simulink model "das_model"  (R2026a)
settings: Solver=FixedStepDiscrete  StopTime=T_sim  FixedStep=Ts_slow
InitFcn:
  | addpath(fullfile(fileparts(get_param(bdroot,'FileName')),'..','scripts')); p = otdr_params(); das_init
undefined symbols (not defined in the file): att, B_cell, f_v, g_cir, g_edfa, g_vib, k_lo, k_sig, Ns, p, p_frame, P_laser, Phi0, r, R_pd, sigma_n_coh, sigma_n_dd, Ts_slow, var_phL
settings Model: Creator=aljou  LastModifiedBy=aljou

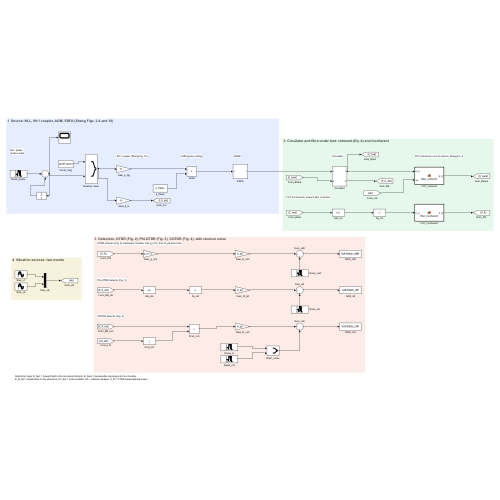
[thumbnail: Simulink's stored preview of the top-level diagram]
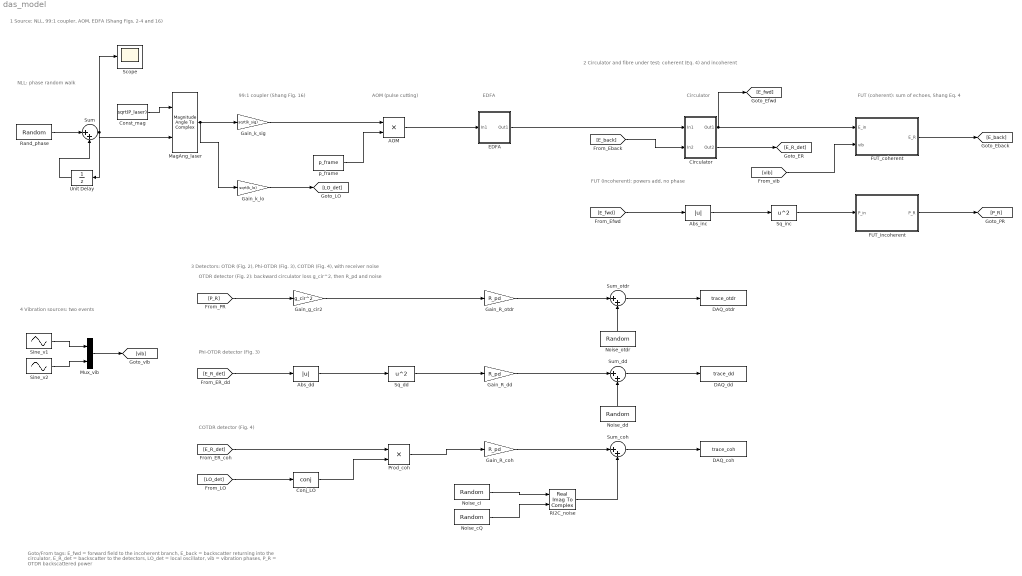
== system das_model ==
  note: NLL: phase
      | random walk
  note: 99:1 coupler (Shang Fig. 16)
  note: AOM (pulse cutting)
  note: EDFA
  note: Circulator
  note: FUT (coherent): sum of echoes, Shang Eq. 4
  note: FUT (incoherent): powers add, no phase
  note: OTDR detector (Fig. 2): backward circulator loss g_cir^2, then R_pd and noise
  note: Phi-OTDR detector (Fig. 3)
  note: COTDR detector (Fig. 4)
  note: Goto/From tags: E_fwd = forward field to the incoherent branch, E_back = backscatter returning into the circulator,
      | E_R_det = backscatter to the detectors, LO_det = local oscillator, vib = vibration phases, P_R = OTDR backscattered power
  note: 1 Source: NLL, 99:1 coupler, AOM, EDFA (Shang Figs. 2-4 and 16)
  note: 2 Circulator and fibre under test: coherent (Eq. 4) and incoherent
  note: 3 Detectors: OTDR (Fig. 2), Phi-OTDR (Fig. 3), COTDR (Fig. 4), with receiver noise
  note: 4 Vibration sources: two events
  AOM : Product  Inputs=**
  Abs_dd : Abs  SaturateOnIntegerOverflow=off
  Abs_inc : Abs  SaturateOnIntegerOverflow=off
  Circulator : Subsystem
  Conj_LO : Math  Operator=conj
  Const_mag : Constant  Value=sqrt(P_laser)  SampleTime=Ts_slow
  DAQ_coh : ToWorkspace  VariableName=trace_coh  SampleTime=Ts_slow
  DAQ_dd : ToWorkspace  VariableName=trace_dd  SampleTime=Ts_slow
  DAQ_otdr : ToWorkspace  VariableName=trace_otdr  SampleTime=Ts_slow
  EDFA : Subsystem
  FUT_coherent : MATLAB Function  TreatAsAtomicUnit=on
  FUT_incoherent : MATLAB Function  TreatAsAtomicUnit=on
  Gain_R_coh : Gain  Gain=R_pd
  Gain_R_dd : Gain  Gain=R_pd
  Gain_R_otdr : Gain  Gain=R_pd
  Gain_g_cir2 : Gain  Gain=g_cir^2
  Gain_k_lo : Gain  Gain=sqrt(k_lo)
  Gain_k_sig : Gain  Gain=sqrt(k_sig)
  MagAng_laser : MagnitudeAngleToComplex
  Mux_vib : Mux  Inputs=2
  Noise_cI : RandomNumber  Mean=zeros(Ns,1)  Variance=sigma_n_coh^2  Seed=p.seed_noise(3)+(1:Ns).'  SampleTime=Ts_slow  VectorParams1D=off
  Noise_cQ : RandomNumber  Mean=zeros(Ns,1)  Variance=sigma_n_coh^2  Seed=p.seed_noise(4)+(1:Ns).'  SampleTime=Ts_slow  VectorParams1D=off
  Noise_dd : RandomNumber  Mean=zeros(Ns,1)  Variance=sigma_n_dd^2  Seed=p.seed_noise(2)+(1:Ns).'  SampleTime=Ts_slow  VectorParams1D=off
  Noise_otdr : RandomNumber  Mean=zeros(Ns,1)  Variance=sigma_n_dd^2  Seed=p.seed_noise(1)+(1:Ns).'  SampleTime=Ts_slow  VectorParams1D=off
  Prod_coh : Product  Inputs=**
  RI2C_noise : RealImagToComplex
  Rand_phase : RandomNumber  Variance=var_phL  Seed=p.seed_laser  SampleTime=Ts_slow
  Scope : Scope
      settings: ActiveDisplayYMinimum=-56.44665138784287  ActiveDisplayYMaximum=140.2998758824863
  Sine_v1 : Sin  Amplitude=Phi0(1)  Frequency=2*pi*f_v(1)  Phase=p.sine_phase  SampleTime=Ts_slow
  Sine_v2 : Sin  Amplitude=Phi0(2)  Frequency=2*pi*f_v(2)  Phase=p.sine_phase  SampleTime=Ts_slow
  Sq_dd : Math  Operator=square
  Sq_inc : Math  Operator=square
  Sum : Sum  Inputs=|++
  Sum_coh : Sum  Inputs=|++
  Sum_dd : Sum  Inputs=|++
  Sum_otdr : Sum  Inputs=|++
  Unit Delay : UnitDelay  SampleTime=Ts_slow
  p_frame : Constant  Value=p_frame  VectorParams1D=off  SampleTime=Ts_slow
  wires:
  Rand_phase/1 -> Sum/1
  Sum/1 -> Unit Delay/1, MagAng_laser/2, Scope/1
  Unit Delay/1 -> Sum/2
  Const_mag/1 -> MagAng_laser/1
  MagAng_laser/1 -> Gain_k_sig/1, Gain_k_lo/1
  Gain_k_lo/1 -> [LO_det]
  Gain_k_sig/1 -> AOM/1
  p_frame/1 -> AOM/2
  AOM/1 -> EDFA/1(In1)
  EDFA/1(Out1) -> Circulator/1(In1)
  [E_back] -> Circulator/2(In2)
  Circulator/2(Out2) -> [E_R_det]
  Circulator/1(Out1) -> FUT_coherent/1(E_in), [E_fwd]
  [vib] -> FUT_coherent/2(vib)
  FUT_coherent/1(E_R) -> [E_back]
  [E_fwd] -> Abs_inc/1
  Abs_inc/1 -> Sq_inc/1
  Sq_inc/1 -> FUT_incoherent/1(P_in)
  FUT_incoherent/1(P_R) -> [P_R]
  Sine_v1/1 -> Mux_vib/1
  Sine_v2/1 -> Mux_vib/2
  Mux_vib/1 -> [vib]
  [P_R] -> Gain_g_cir2/1
  Gain_g_cir2/1 -> Gain_R_otdr/1
  Gain_R_otdr/1 -> Sum_otdr/1
  Sum_otdr/1 -> DAQ_otdr/1
  Noise_otdr/1 -> Sum_otdr/2
  [E_R_det] -> Abs_dd/1
  Abs_dd/1 -> Sq_dd/1
  Sq_dd/1 -> Gain_R_dd/1
  Gain_R_dd/1 -> Sum_dd/1
  Sum_dd/1 -> DAQ_dd/1
  Noise_dd/1 -> Sum_dd/2
  [E_R_det] -> Prod_coh/1
  [LO_det] -> Conj_LO/1
  Conj_LO/1 -> Prod_coh/2
  Prod_coh/1 -> Gain_R_coh/1
  Gain_R_coh/1 -> Sum_coh/1
  Sum_coh/1 -> DAQ_coh/1
  Noise_cI/1 -> RI2C_noise/1
  Noise_cQ/1 -> RI2C_noise/2
  RI2C_noise/1 -> Sum_coh/2

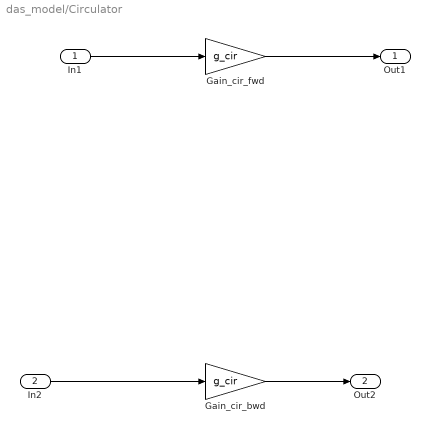
== system das_model/Circulator ==
  In1 : Inport
  In2 : Inport  Port=2
  Gain_cir_bwd : Gain  Gain=g_cir
  Gain_cir_fwd : Gain  Gain=g_cir
  Out1 : Outport
  Out2 : Outport  Port=2
  wires:
  In2/1 -> Gain_cir_bwd/1
  Gain_cir_fwd/1 -> Out1/1
  Gain_cir_bwd/1 -> Out2/1
  In1/1 -> Gain_cir_fwd/1

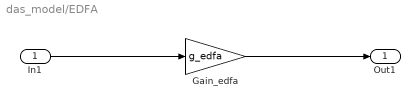
== system das_model/EDFA ==
  In1 : Inport
  Gain_edfa : Gain  Gain=g_edfa
  Out1 : Outport
  wires:
  Gain_edfa/1 -> Out1/1
  In1/1 -> Gain_edfa/1

== matlab function das_model/FUT_incoherent ==
  data: P_in input; P_R output; att parameter; B_cell parameter
function P_R = fiber_incoherent(P_in, att, B_cell)
%FIBER_INCOHERENT  FUT block for conventional OTDR (low-coherence source).
%  Paste this into a MATLAB Function block named "FUT (incoherent)".
%    P_in   : input,  Size [Ns 1], real   (probe POWER frame = |E|^2)
%    B_cell : PARAMETER (scalar)          (backscattered power fraction per cell)
%    att    : PARAMETER (Nz x 1)          (same as the coherent block)
%    P_R    : output, Size [Ns 1], real   (backscattered POWER)
%
%  With a low-coherence source the echoes do not interfere: powers add, not
%  fields. The vibration phase therefore has no effect on the trace — this is
%  exactly why conventional OTDR cannot sense vibration (Shang 2022, Sec. 2.2).
%
%  Change vs the original: the power response uses the AVERAGE scattering power
%  B_cell instead of the random |r|^2. A low-coherence source averages the
%  speckle away, so the trace is a smooth line (slope = 2*alpha).

h   = B_cell .* att.^2;                  % power impulse response (round trip)
y   = conv(P_in, h);
P_R = y(1:numel(P_in));
end

== matlab function das_model/FUT_coherent ==
  data: E_in input; E_R output; vib input; r parameter; g_vib parameter; att parameter
function E_R = fiber_coherent(E_in, vib, r, g_vib, att)
%FIBER_COHERENT  FUT block for Phi-OTDR and COTDR (coherent laser).
%  Paste this into a MATLAB Function block named "FUT (coherent)".
%  Ports and Data Manager settings (set Size explicitly, it avoids dimension errors):
%    E_in  : input,  Size [Ns 1], Complexity complex  (probe frame after EDFA + circulator)
%    vib   : input,  Size [K 1] (or [1 K] from the Mux), real  (vibration phase of each event)
%    r     : PARAMETER (Nz x 1 complex), att : PARAMETER (Nz x 1), g_vib : PARAMETER (Nz x K)
%    E_R   : output, Size [Ns 1], Complexity complex
%
%  Model (Shang 2022, Eq. 4): the received field is the sum of the echoes of
%  all scatterers. Each fibre cell is one scatterer, delayed by its round trip
%  (one sample per cell), so the sum becomes a convolution of the probe with
%  the fibre impulse response h.  A vibration adds a phase to every cell at
%  and beyond the disturbed section.

phi = g_vib * vib(:);                    % Nz x 1 extra phase [rad]  (vib(:) forces a column)
h   = r .* att .* exp(1j*phi);           % fibre impulse response
y   = conv(E_in, h);                     % coherent sum of all echoes
E_R = y(1:numel(E_in));
end
